simulink model "Pole_placement_simulink"  (R2023b)
settings: Solver=VariableStepAuto  StartTime=0.0  StopTime=50  RelTol=1e-3
values from neighbouring files (symbols this model uses):
  A = [0 1 0 0;32.79 0 6.625 0;0 0 0 1;-67.38 0 -8.92 0]    [Pole_placement.m]
  Aobs = A-(L'*C)    [Pole_placement.m]
  B = [0 0; 4.65 -7.94;0 0;-7.94 27.27]    [Pole_placement.m]
  Bobs = [B L']    [Pole_placement.m]
  C = [1 0 0 0;0 0 1 0]    [Pole_placement.m]
  Cobs = eye(4)    [Pole_placement.m]
  D = zeros(2,2)    [Pole_placement.m]
  Dobs = zeros(4)    [Pole_placement.m]
  gainMatrix = (dcgain(tfMatrixPos))^-1    [Pole_placement.m]
  gainMatrixITAE = (dcgain(tfMatrixPosITAE))^-1    [Pole_placement.m]
  K = place(A,B,pcc)    [Pole_placement.m]
  Kfinal = place(Aaug,Baug,pcci)    [Pole_placement.m]
  KiITAE = place(Aaug,Baug,piITAE)    [Pole_placement.m]
  KITAE = place(A,B,pITAE)    [Pole_placement.m]
settings Model: Creator=Giammo  LastModifiedBy=Giammo

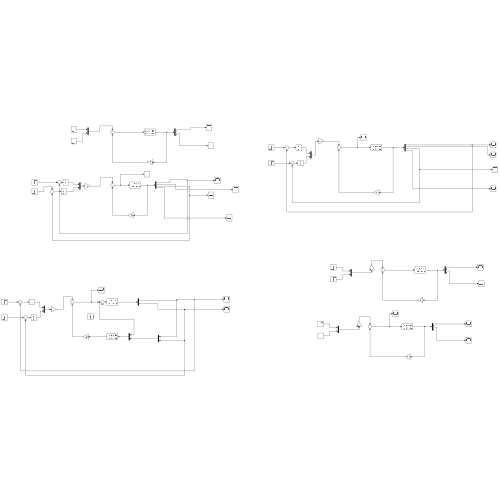
[thumbnail: Simulink's stored preview of the top-level diagram]
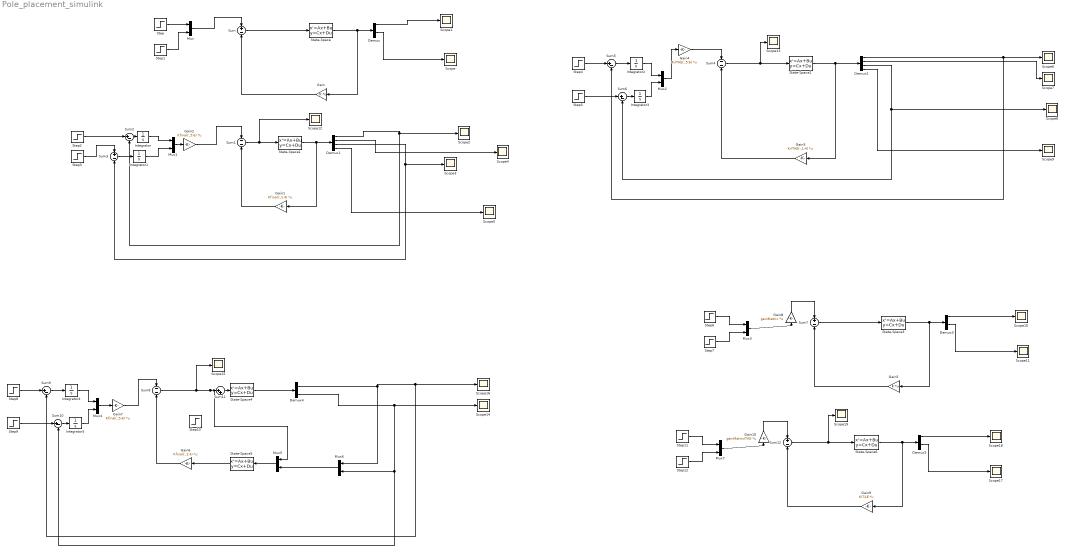
== system Pole_placement_simulink ==
  Demux{,1..3,5} (5 alike) : Demux
  Demux4 : Demux  Outputs=2
  Gain : Gain  Gain=K  Multiplication=Matrix(K*u)
  Gain1 : Gain  Gain=Kfinal(:,1:4)  Multiplication=Matrix(K*u)
  Gain10 : Gain  Gain=gainMatrixITAE  Multiplication=Matrix(K*u)
  Gain2 : Gain  Gain=Kfinal(:,5:6)  Multiplication=Matrix(K*u)
  Gain3 : Gain  Gain=KiITAE(:,1:4)  Multiplication=Matrix(K*u)
  Gain4 : Gain  Gain=KiITAE(:,5:6)  Multiplication=Matrix(K*u)
  Gain5 : Gain  Gain=K  Multiplication=Matrix(K*u)
  Gain6 : Gain  Gain=Kfinal(:,1:4)  Multiplication=Matrix(K*u)
  Gain7 : Gain  Gain=Kfinal(:,5:6)  Multiplication=Matrix(K*u)
  Gain8 : Gain  Gain=gainMatrix  Multiplication=Matrix(K*u)
  Gain9 : Gain  Gain=KITAE  Multiplication=Matrix(K*u)
  Integrator{,1..5} (6 alike) : Integrator
  Mux{,1..7} (8 alike) : Mux  Inputs=2
  Scope{,1..19} (20 alike) : Scope
  State-Space : StateSpace  A=A  B=B  C=eye(4)  D=zeros(4,2)  InitialCondition=[0;0;0;0]
  State-Space{1..3,6} (4 alike) : StateSpace  A=A  B=B  C=eye(4)  D=zeros(4,2)  InitialCondition=0
  State-Space4 : StateSpace  A=A  B=B  C=C  D=D  InitialCondition=0
  State-Space5 : StateSpace  A=Aobs  B=Bobs  C=Cobs  D=Dobs  InitialCondition=[0.2;0;0.2;0]
  Step{,1..9} (10 alike) : Step  After=0.26  SampleTime=0
  Step10 : Step  SampleTime=0
  Step11 : Step  SampleTime=0
  Step12 : Step  SampleTime=0
  Sum{,3,7,12} (4 alike) : Sum  Inputs=+-
  Sum1 : Sum  Inputs=--
  Sum{2,5..6,9..10} (5 alike) : Sum  Inputs=|+-
  Sum11 : Sum  Inputs=|++
  Sum4 : Sum  Inputs=--
  Sum8 : Sum  Inputs=--
  wires:
  State-Space/1 -> Gain/1, Demux/1
  Demux/1 -> Scope1/1
  Demux/3 -> Scope/1
  Gain/1 -> Sum/2
  Sum/1 -> State-Space/1
  Step/1 -> Mux/1
  Step1/1 -> Mux/2
  Mux/1 -> Sum/1
  State-Space1/1 -> Gain1/1, Demux1/1
  Sum1/1 -> State-Space1/1, Scope12/1
  Gain1/1 -> Sum1/2
  Step2/1 -> Sum2/1
  Step3/1 -> Sum3/1
  Demux1/1 -> Sum2/2, Scope2/1
  Demux1/3 -> Sum3/2, Scope3/1
  Sum3/1 -> Integrator1/1
  Sum2/1 -> Integrator/1
  Integrator/1 -> Mux1/1
  Integrator1/1 -> Mux1/2
  Mux1/1 -> Gain2/1
  Gain2/1 -> Sum1/1
  Demux1/2 -> Scope4/1
  Demux1/4 -> Scope5/1
  Sum5/1 -> Integrator2/1
  Demux2/4 -> Scope9/1
  Integrator2/1 -> Mux2/1
  Step5/1 -> Sum6/1
  Mux2/1 -> Gain4/1
  Sum6/1 -> Integrator3/1
  Sum4/1 -> Scope13/1, State-Space2/1
  Gain3/1 -> Sum4/2
  Integrator3/1 -> Mux2/2
  Step4/1 -> Sum5/1
  Gain4/1 -> Sum4/1
  Demux2/2 -> Scope7/1
  State-Space2/1 -> Gain3/1, Demux2/1
  Demux2/1 -> Scope6/1, Sum5/2
  Demux3/3 -> Scope11/1
  State-Space3/1 -> Gain5/1, Demux3/1
  Mux3/1 -> Gain8/1
  Sum7/1 -> State-Space3/1
  Gain5/1 -> Sum7/2
  Demux2/3 -> Scope8/1, Sum6/2
  Step6/1 -> Mux3/1
  Step7/1 -> Mux3/2
  Gain8/1 -> Sum7/1
  Demux3/1 -> Scope10/1
  Demux5/1 -> Scope18/1
  Step11/1 -> Mux7/1
  Mux7/1 -> Gain10/1
  Sum12/1 -> Scope19/1, State-Space6/1
  Gain10/1 -> Sum12/1
  Demux5/3 -> Scope17/1
  Step12/1 -> Mux7/2
  State-Space6/1 -> Gain9/1, Demux5/1
  Gain9/1 -> Sum12/2
  Sum9/1 -> Integrator4/1
  Step8/1 -> Sum9/1
  Gain6/1 -> Sum8/2
  Mux4/1 -> Gain7/1
  Integrator5/1 -> Mux4/2
  Mux6/1 -> Mux5/2
  Sum11/1 -> State-Space4/1
  Sum8/1 -> Scope15/1, Mux5/1, Sum11/1
  Step9/1 -> Sum10/1
  Gain7/1 -> Sum8/1
  State-Space4/1 -> Demux4/1
  State-Space5/1 -> Gain6/1
  Mux5/1 -> State-Space5/1
  Integrator4/1 -> Mux4/1
  Sum10/1 -> Integrator5/1
  Demux4/1 -> Scope16/1, Sum9/2, Mux6/1
  Demux4/2 -> Sum10/2, Mux6/2, Scope14/1
